simulink model "stabilizer_bar_step35g"  (R2023a)
settings: Solver=ode4  StartTime=0  StopTime=40  FixedStep=Ts_plant  MaxStep=0.001  RelTol=1e-3
InitFcn:
  | run(fullfile(fileparts(get_param(bdroot,'FileName')),'a001_step35g_initialize.m'));
values from neighbouring files (symbols this model uses):
  cycle_cfg = jsondecode(fileread(fullfile(repair_root,'repair_support','repair_cycle_bank.json')))    [a001_step35g_initialize.m]
  entry_cfg = rmfield(entry_bank_source,{'labels','source_hashes','note','source_par_sha256'})    [a001_step35g_initialize.m]
  path_geometry = repair_build_geometry(path_cfg)    [a001_step35g_initialize.m]
  path_Q = [10,0,0;0,10,0;0,0,2]    [a001_step35g_initialize.m]
  path_R = [100,0,0;0,100,0;0,0,10]    [a001_step35g_initialize.m]
  repair_cfg = struct    [a001_step35g_initialize.m]
  repair_simfile = aux_case_cfg.simfile_path    [a001_step35g_initialize.m]
  stadium_cfg = struct('disabled',1)    [a001_step35g_initialize.m]
  state_cfg = profile_cfg.state_protocol    [a001_step35g_initialize.m]
  Ts = 0.01    [a001_step35g_initialize.m]
  Ts_plant = 0.0005    [a001_step35g_initialize.m]
undefined symbols (not defined in the file or in its folder): path_cfg
(part 2 of 2)

== matlab function stabilizer_bar_step35g/路径跟踪层/ContinuousProjection ==
  settings: updateMethod=DISCRETE  sampleTime=Ts
  data: X input; ey output size=1; Y input; psi input; beta input; alignment input size=[3 1]; DeltaChi output size=1; kappa output size=1; diag_project output size=[2 1]; path_geometry parameter; path_cfg parameter
function [ey,DeltaChi,kappa,diag_project] = path_projection(X,Y,psi,beta,alignment,path_geometry,path_cfg)
%#codegen
% 连续Frenet投影：只沿上一个弧长邻域迭代，弧长不取模存储，跨圈不跳点。
% ey为路径左侧正；DeltaChi为实际速度方向psi+beta与投影切向之差。
% 该投影用于式4.10；LQR仍跟踪时间索引参考，二者用途明确区分。
if path_cfg.feedback_enabled==0,ey=0;DeltaChi=0;kappa=0;diag_project=zeros(2,1);return;end
persistent s_prev
if isempty(s_prev),s_prev=0;end
c=cos(alignment(3));sn=sin(alignment(3));
dx=X-alignment(1);dy=Y-alignment(2);
x=c*dx+sn*dy;y=-sn*dx+c*dy;
s=s_prev;
% 牛顿投影的分母即1-kappa*ey；失效时停止，不夹紧分母。
for it=1:12
    [px,py,chi,k]=geometry(s,path_geometry,path_cfg);
    ex=x-px;ey0=y-py;
    lateral=-sin(chi)*ex+cos(chi)*ey0;
    den=1-k*lateral;
    % 分母状态只记录，不触发外加仿真停止。
    ds=(cos(chi)*ex+sin(chi)*ey0)/den;
    % 有界迭代步只用于局部求根，不能切换到全局另一段路径。
    s=s+ds;
    % 投影点跳变由路径误差和CarSim响应体现，不用Assert截断仿真。
    if abs(ds)<1e-7,break;end
end
[px,py,chi,kappa]=geometry(s,path_geometry,path_cfg);
ey=-sin(chi)*(x-px)+cos(chi)*(y-py);
tangential=cos(chi)*(x-px)+sin(chi)*(y-py);
% 切向投影残差保留在后续诊断中。
DeltaChi=atan2(sin(psi+beta-alignment(3)-chi),cos(psi+beta-alignment(3)-chi));
den=1-kappa*ey;
% 分母状态只记录，不触发外加仿真停止。
s_prev=s;diag_project=[s;den];
end
function [x,y,chi,k]=geometry(s,table,cfg)
if (cfg.mode==4 || cfg.mode==5),q=mod(s,cfg.length);else,q=s;end
[x,y,chi]=sample_geometry(q,table,cfg);
[k,~,~,~,~]=repair_path_profile(s,cfg);
end
function [x,y,chi]=sample_geometry(q,table,cfg)
% 均匀节点三次Hermite位置插值，切向由同一曲率积分生成。
ds=table(2,1)-table(1,1);j=min(max(floor(q/ds)+1,1),size(table,1)-1);
h=table(j+1,1)-table(j,1);u=(q-table(j,1))/h;
h00=2*u^3-3*u^2+1;h10=u^3-2*u^2+u;h01=-2*u^3+3*u^2;h11=u^3-u^2;
x=h00*table(j,2)+h10*h*cos(table(j,4))+h01*table(j+1,2)+h11*h*cos(table(j+1,4));
y=h00*table(j,3)+h10*h*sin(table(j,4))+h01*table(j+1,3)+h11*h*sin(table(j+1,4));
[~,~,~,~,chi]=repair_path_profile(q,cfg);
end

function [k,bw,dbds,stage,chi]=repair_path_profile(s,cfg)
% 曲率与侧偏角分别生成；chi是曲率对弧长的解析积分。
% mode=1入漂维持，2同步退出，3先恢复beta再退出，4原操场，5提前恢复beta操场。
L=cfg.transition;R=cfg.R;C=cfg.plateau;
% 普通轨迹：stage=1直线、2入弯、3恒曲率、4出弯、5末直线。
% 曲率与漂移权重独立；mode=6始终bw=0，不能只把beta设零。
if cfg.mode==6
 q=s-cfg.straight;bw=0;dbds=0;
 if q<=0,k=0;chi=0;stage=1;
 elseif q<L
  u=q/L;[h,~]=smooth(u);k=h/R;chi=L/R*primitive(u);stage=2;
 elseif q<L+C,k=1/R;chi=(q-L/2)/R;stage=3;
 elseif q<2*L+C
  u=(q-L-C)/L;[h,~]=smooth(u);k=(1-h)/R;chi=(L/2+C+L*(u-primitive(u)))/R;stage=4;
 else,k=0;chi=(L+C)/R;stage=5;end
 return;
end
if cfg.mode==4 || cfg.mode==5
 q=mod(s,cfg.half)-cfg.straight;half=floor(s/cfg.half);
 if q<=0,k=0;bw=0;dbds=0;stage=1;theta=0;
 elseif q<L
  u=q/L;[bw,db]=smooth(u);dbds=db/L;k=bw/R;stage=2;theta=L/R*primitive(u);
 elseif q<L+C
  k=1/R;bw=1;dbds=0;stage=3;theta=(q-L/2)/R;
  if cfg.mode==5 && q>L+C-L
   u=(q-(L+C-L))/L;[z,dz]=smooth(u);bw=1-z;dbds=-dz/L;stage=4;
  end
 else
  u=min((q-L-C)/L,1);[z,dz]=smooth(u);k=(1-z)/R;
  if cfg.mode==4,bw=1-z;dbds=-dz/L;else,bw=0;dbds=0;end
  stage=4;theta=(L/2+C+L*(u-primitive(u)))/R;
 end
 chi=pi*half+theta;stage=stage+4*mod(half,2);return;
end
% 入漂维持允许曲率与侧偏的建立长度/起点不同；chi仍只由曲率积分确定。
if cfg.mode==1
 q=s-cfg.straight;u=min(max(q/cfg.transition,0),1);[hk,~]=smooth(u);k=hk/cfg.R;
 if q<=0,chi=0;elseif q<cfg.transition,chi=cfg.transition/cfg.R*primitive(u);else,chi=(q-cfg.transition/2)/cfg.R;end
 v=min(max((q-cfg.beta_delay)/cfg.beta_transition,0),1);[bw,db]=smooth(v);dbds=db/cfg.beta_transition;
 if q<=0,stage=1;elseif u<1||v<1,stage=2;else,stage=3;end
 return;
end
q=s-cfg.straight;
if q<=0,k=0;bw=0;dbds=0;stage=1;chi=0;return;end
if q<L
 u=q/L;[bw,db]=smooth(u);dbds=db/L;k=bw/R;stage=2;chi=L/R*primitive(u);return;
end
k=1/R;bw=1;dbds=0;stage=3;chi=(q-L/2)/R;
if cfg.mode==1,return;end
% 独立退出站点由已通过3s稳态门槛的前置试验给出，不猜测稳定起点。
e=s-cfg.exit_s;if e<0,return;end
if cfg.mode==2
 u=min(e/L,1);[z,dz]=smooth(u);k=(1-z)/R;bw=1-z;dbds=-dz/L;
 chi=(cfg.exit_s-cfg.straight-L/2+L*(u-primitive(u)))/R;stage=4;
else
 u=min(e/L,1);[z,dz]=smooth(u);bw=1-z;dbds=-dz/L;stage=4;
 if e>=L
  z2=min((e-L)/L,1);[h,~]=smooth(z2);k=(1-h)/R;
  chi=(cfg.exit_s+L-cfg.straight-L/2+L*(z2-primitive(z2)))/R;stage=5;
 end
end
end
function [h,dh]=smooth(u)
h=10*u^3-15*u^4+6*u^5;dh=30*u^2*(1-u)^2;
end
function v=primitive(u)
v=2.5*u^4-3*u^5+u^6;
end

== matlab function stabilizer_bar_step35g/CarSimInterface/FrontWheelActuator ==
  settings: updateMethod=DISCRETE  sampleTime=Ts_plant
  data: target input; left output; right output; left_rate output; right_rate output; diag output size=[6 1]; repair_cfg parameter
function [left,right,left_rate,right_rate,diag] = steer_direct(target,repair_cfg)
% 直接前轮输入，不叠加外部转角幅值或速率限制；角速度同步记录指令变化率。
persistent previous
if isempty(previous),previous=0;end
angle=target(1);
if repair_cfg.entry_mode==1,limit=repair_cfg.entry_steer_rate*repair_cfg.Ts_plant;angle=min(max(angle,previous-limit),previous+limit);end
rate=(angle-previous)/repair_cfg.Ts_plant;previous=angle;
left=angle*180/pi;right=left;left_rate=rate*180/pi;right_rate=left_rate;
diag=[angle;angle;angle;rate;0;0];
end

== matlab function stabilizer_bar_step35g/CarSimInterface/InterfaceTestSelector ==
  settings: updateMethod=DISCRETE  sampleTime=Ts_plant
  data: command input size=[8 1]; u output size=[8 1]; t input; repair_interface_test parameter
function u=interface_selector(command,t,repair_interface_test)
% 仅在显式接口验证中产生2deg、10deg/s分段线性转角；其余时候透传。
u=command;
if repair_interface_test==0,return;end
knots=[0,.4,.6,.9,1.1,1.3,1.6,1.8,2,2.3,2.7,3,3.2,3.6];
left=[0,0,2,2,0,0,0,0,2,2,-2,-2,0,0];right=[0,0,0,0,0,-2,-2,0,2,2,-2,-2,0,0];
j=1;for k=1:13,if t>=knots(k),j=k;end;end
q=min(max((t-knots(j))/(knots(j+1)-knots(j)),0),1);
lr=(left(j+1)-left(j))/(knots(j+1)-knots(j));rr=(right(j+1)-right(j))/(knots(j+1)-knots(j));
u=[left(j)+q*(left(j+1)-left(j));right(j)+q*(right(j+1)-right(j));lr;rr;0;0;0;0];
end

== matlab function stabilizer_bar_step35g/StageStop ==
  settings: updateMethod=DISCRETE  sampleTime=Ts
  data: valid input; stop output; plant input size=[50 1]; repair_interface_test parameter
function stop=stage_stop(valid,plant,repair_interface_test)
% 仅保留信号记录；候选、轮荷、查表告警不再触发自定义Stop Simulation。
stop=0;
end

== matlab function stabilizer_bar_step35g/路径跟踪层/ReferenceAlignment ==
  settings: updateMethod=DISCRETE  sampleTime=Ts
  data: t input; ref output size=[14 1]; X input; Y input; psi input; V input; alignment output size=[3 1]; path_geometry parameter; path_cfg parameter
function [ref,alignment]=stadium_reference(t,X,Y,psi,V,path_geometry,path_cfg)
% 统一工况参考：初始实际质心对齐；入漂维持与两种退出独立选择。
% ref的14项接口与现有路径层保持一致，所有角度为rad。
persistent origin initial_speed
if isempty(origin),origin=[X;Y;psi];initial_speed=V;end
alignment=origin;T=path_cfg.ramp_time;u=min(max(t/T,0),1);H=10*u^3-15*u^4+6*u^5;
Vr=initial_speed+(path_cfg.V-initial_speed)*H;
if t<=T,s=initial_speed*t+(path_cfg.V-initial_speed)*T*(2.5*u^4-3*u^5+u^6);
else,s=(initial_speed+path_cfg.V)*T/2+path_cfg.V*(t-T);end
[k,bw,dbds,stage,chi]=repair_path_profile(s,path_cfg);
beta=path_cfg.beta*bw;bdot=path_cfg.beta*dbds*Vr;
if (path_cfg.mode==4 || path_cfg.mode==5),q=mod(s,path_cfg.length);lap=floor(s/path_cfg.length);else,q=s;lap=0;end
[x,y,~]=sample_geometry(q,path_geometry,path_cfg);
c=cos(origin(3));sn=sin(origin(3));chi=chi+origin(3);
ref=[origin(1)+c*x-sn*y;origin(2)+sn*x+c*y;chi-beta;Vr*cos(beta);Vr*sin(beta); ...
 k*Vr-bdot;Vr;beta;k;bw;stage;lap;s;chi];
end

function [x,y,chi]=sample_geometry(q,table,cfg)
% 均匀节点三次Hermite位置插值，切向由同一曲率积分生成。
ds=table(2,1)-table(1,1);j=min(max(floor(q/ds)+1,1),size(table,1)-1);
h=table(j+1,1)-table(j,1);u=(q-table(j,1))/h;
h00=2*u^3-3*u^2+1;h10=u^3-2*u^2+u;h01=-2*u^3+3*u^2;h11=u^3-u^2;
x=h00*table(j,2)+h10*h*cos(table(j,4))+h01*table(j+1,2)+h11*h*cos(table(j+1,4));
y=h00*table(j,3)+h10*h*sin(table(j,4))+h01*table(j+1,3)+h11*h*sin(table(j+1,4));
[~,~,~,~,chi]=repair_path_profile(q,cfg);
end

function [k,bw,dbds,stage,chi]=repair_path_profile(s,cfg)
% 曲率与侧偏角分别生成；chi是曲率对弧长的解析积分。
% mode=1入漂维持，2同步退出，3先恢复beta再退出，4原操场，5提前恢复beta操场。
L=cfg.transition;R=cfg.R;C=cfg.plateau;
% 普通轨迹：stage=1直线、2入弯、3恒曲率、4出弯、5末直线。
% 曲率与漂移权重独立；mode=6始终bw=0，不能只把beta设零。
if cfg.mode==6
 q=s-cfg.straight;bw=0;dbds=0;
 if q<=0,k=0;chi=0;stage=1;
 elseif q<L
  u=q/L;[h,~]=smooth(u);k=h/R;chi=L/R*primitive(u);stage=2;
 elseif q<L+C,k=1/R;chi=(q-L/2)/R;stage=3;
 elseif q<2*L+C
  u=(q-L-C)/L;[h,~]=smooth(u);k=(1-h)/R;chi=(L/2+C+L*(u-primitive(u)))/R;stage=4;
 else,k=0;chi=(L+C)/R;stage=5;end
 return;
end
if cfg.mode==4 || cfg.mode==5
 q=mod(s,cfg.half)-cfg.straight;half=floor(s/cfg.half);
 if q<=0,k=0;bw=0;dbds=0;stage=1;theta=0;
 elseif q<L
  u=q/L;[bw,db]=smooth(u);dbds=db/L;k=bw/R;stage=2;theta=L/R*primitive(u);
 elseif q<L+C
  k=1/R;bw=1;dbds=0;stage=3;theta=(q-L/2)/R;
  if cfg.mode==5 && q>L+C-L
   u=(q-(L+C-L))/L;[z,dz]=smooth(u);bw=1-z;dbds=-dz/L;stage=4;
  end
 else
  u=min((q-L-C)/L,1);[z,dz]=smooth(u);k=(1-z)/R;
  if cfg.mode==4,bw=1-z;dbds=-dz/L;else,bw=0;dbds=0;end
  stage=4;theta=(L/2+C+L*(u-primitive(u)))/R;
 end
 chi=pi*half+theta;stage=stage+4*mod(half,2);return;
end
% 入漂维持允许曲率与侧偏的建立长度/起点不同；chi仍只由曲率积分确定。
if cfg.mode==1
 q=s-cfg.straight;u=min(max(q/cfg.transition,0),1);[hk,~]=smooth(u);k=hk/cfg.R;
 if q<=0,chi=0;elseif q<cfg.transition,chi=cfg.transition/cfg.R*primitive(u);else,chi=(q-cfg.transition/2)/cfg.R;end
 v=min(max((q-cfg.beta_delay)/cfg.beta_transition,0),1);[bw,db]=smooth(v);dbds=db/cfg.beta_transition;
 if q<=0,stage=1;elseif u<1||v<1,stage=2;else,stage=3;end
 return;
end
q=s-cfg.straight;
if q<=0,k=0;bw=0;dbds=0;stage=1;chi=0;return;end
if q<L
 u=q/L;[bw,db]=smooth(u);dbds=db/L;k=bw/R;stage=2;chi=L/R*primitive(u);return;
end
k=1/R;bw=1;dbds=0;stage=3;chi=(q-L/2)/R;
if cfg.mode==1,return;end
% 独立退出站点由已通过3s稳态门槛的前置试验给出，不猜测稳定起点。
e=s-cfg.exit_s;if e<0,return;end
if cfg.mode==2
 u=min(e/L,1);[z,dz]=smooth(u);k=(1-z)/R;bw=1-z;dbds=-dz/L;
 chi=(cfg.exit_s-cfg.straight-L/2+L*(u-primitive(u)))/R;stage=4;
else
 u=min(e/L,1);[z,dz]=smooth(u);bw=1-z;dbds=-dz/L;stage=4;
 if e>=L
  z2=min((e-L)/L,1);[h,~]=smooth(z2);k=(1-h)/R;
  chi=(cfg.exit_s+L-cfg.straight-L/2+L*(z2-primitive(z2)))/R;stage=5;
 end
end
end
function [h,dh]=smooth(u)
h=10*u^3-15*u^4+6*u^5;dh=30*u^2*(1-u)^2;
end
function v=primitive(u)
v=2.5*u^4-3*u^5+u^6;
end

== matlab function stabilizer_bar_step35g/EntryLocalMode/EntryLocalControl ==
  settings: updateMethod=DISCRETE  sampleTime=Ts
  data: y input size=[50 1]; command output size=[5 1]; t input; diag output size=[70 1]; entry_cfg parameter; repair_cfg parameter; cycle_diag output size=[16 1]; cycle_cfg parameter; stadium_packet input; state_cfg parameter
function [command,diag,cycle_diag]=cycle_control(y,t,entry_cfg,repair_cfg,cycle_cfg,stadium_packet,state_cfg)
%#codegen
% 无路径任务：时间参考→五状态反馈→原公共执行层。这里不读取XY/曲率/方向。
% y是CarSim原50路，轮序FL/FR/RL/RR；stadium_packet现只输送原生600点事件。
% Roll/AVx仅用于原物理接管，K只乘[V,beta,AVz,kappa_f,kappa_r]。
% 进入固定10s维持后不回退/重计；误差与退出门控分开，失败也保留退漂证据。
persistent phase readyTime elapsed entryStart captureTime satTime mixStart holdStart exitStart straightCapture straightMix previousRef refInitialized vprev wprev initialized protection
if isempty(initialized)
 phase=0;readyTime=0;elapsed=0;entryStart=0;captureTime=0;satTime=0;mixStart=0;holdStart=0;exitStart=0;straightCapture=0;straightMix=0;
 previousRef=zeros(7,1);refInitialized=false;vprev=zeros(3,1);wprev=zeros(4,1);initialized=false;protection=false;
end
command=zeros(5,1);diag=zeros(70,1);cycle_diag=zeros(16,1);
Ts=repair_cfg.Ts;Rw=repair_cfg.Rw;Iw=repair_cfg.Iw;
x=[hypot(y(2),y(3))/3.6;y(4)*pi/180;y(5)*pi/180;mean(y(27:28));mean(y(29:30));y(8)*pi/180;y(26)*pi/180];
omega=y(21:24)*pi/30;Fz=y(17:20);last=entry_cfg.nodes(end);
assert(all(isfinite(x))&&all(isfinite(Fz)),'Nonfinite state or wheel load');first=~initialized;
if first,vprev=entry_cfg.normal.v;wprev=omega;initialized=true;end
elapsed=elapsed+Ts;if protection,satTime=satTime+Ts;else,satTime=0;end
inside=all(abs(x-last.x)<=entry_cfg.thresholds)&&all(Fz>0)&&satTime<.2;
progress=0;mix=0;weight=0;holdTime=0;exitProgress=0;substage=0;exitElapsed=0;holdgate=false;prepareFailed=false;
ref=entry_cfg.normal;
% 准备仍由实际直行状态持续1s确定，不使用道路站点或世界坐标。
if phase==0
 ready=abs(x(1)-12)<=.2&&abs(x(2))<=pi/180&&abs(x(3))<=.02;
 if ready,readyTime=readyTime+Ts;else,readyTime=0;end
 ref=mixnode(entry_cfg.normal,entry_cfg.nodes(1),smooth5(t/2));
 if readyTime>=1-1e-9&&elapsed<10,phase=1;entryStart=t;elseif elapsed>=10,prepareFailed=true;end
end
if phase>=1&&phase<=3
 q=max(0,t-entryStart);progress=min(q/state_cfg.entry_reference_s,1);
 % 连续经过节点：预加载复用原公式；其后β一次平滑到−30°。
 % β同时作为原银行的调度坐标，x/v/K/offset共享一个插值比例。
 if q<state_cfg.preload_end_s
  ref=sampleNodes(entry_cfg.nodes(1:7),entry_cfg.grid,smooth5(q/state_cfg.prefix_s));
 else
  h=smooth5((q-state_cfg.preload_end_s)/(state_cfg.entry_reference_s-state_cfg.preload_end_s));
  beta=(1-h)*entry_cfg.nodes(3).x(2)+h*entry_cfg.nodes(9).x(2);
  j=3;
  for k=3:8
   if beta<=entry_cfg.nodes(k).x(2),j=k;end
  end
  f=(beta-entry_cfg.nodes(j).x(2))/(entry_cfg.nodes(j+1).x(2)-entry_cfg.nodes(j).x(2));
  ref=mixnode(entry_cfg.nodes(j),entry_cfg.nodes(j+1),min(max(f,0),1));
 end
 if phase==1
  if inside,captureTime=captureTime+Ts;else,captureTime=0;end
  % 原七项物理接管+独立600原生点确认；原生事件由快采样块生成。
  if q>=state_cfg.entry_reference_s-1e-9&&captureTime>=.3-1e-9&&stadium_packet(1)>0.5
   phase=2;mixStart=t;
  end
 end
 if phase==2
  mix=smooth5((t-mixStart)/state_cfg.handover_s);ref=mixnode(ref,last,mix);
  if t-mixStart>=state_cfg.handover_s-1e-9,phase=3;holdStart=t;end
 end
 if phase==3
  ref=last;mix=1;holdTime=max(0,t-holdStart);
  % 固定窗口满10s即退漂；不以较好的末段RMSE来推迟或重开窗口。
  if holdTime>=state_cfg.maintain_s-1e-9,phase=4;exitStart=t;holdgate=true;end
 end
 weight=mix;
end
if phase>=4
 exitElapsed=max(0,t-exitStart);exitProgress=min(exitElapsed/state_cfg.exit_reference_s,1);
 if exitElapsed<state_cfg.exit_to15_s
  substage=1;ref=mixnode(cycle_cfg.nodes(1),cycle_cfg.nodes(2),smooth5(exitElapsed/state_cfg.exit_to15_s));
 elseif exitElapsed<state_cfg.exit_to15_s+state_cfg.exit_to10_s
  substage=2;ref=mixnode(cycle_cfg.nodes(2),cycle_cfg.nodes(3),smooth5((exitElapsed-state_cfg.exit_to15_s)/state_cfg.exit_to10_s));
 else
  substage=3;q=min((exitElapsed-state_cfg.exit_to15_s-state_cfg.exit_to10_s)/state_cfg.exit_legacy_s,1);
  if q<.5,p=.5*smooth5(2*q);else,p=.5+.5*smooth5(2*q-1);end
  ref=sampleNodes(cycle_cfg.nodes(3:7),cycle_cfg.grid,p);
 end
 normal=cycle_cfg.nodes(end);
 inside=all(abs(x-normal.x)<=cycle_cfg.straight_capture)&&all(Fz>0)&&~protection&&exitProgress>=1-1e-8;
 if inside,straightCapture=straightCapture+Ts;else,straightCapture=0;end
 if phase==4&&straightCapture>=.3-1e-9,phase=5;straightMix=0;end
 if phase==5,straightMix=min(1,straightMix+Ts/.5);if straightMix>=1-1e-9,phase=6;end,end
 weight=0;if phase==5,weight=smooth5(straightMix);elseif phase==6,weight=1;end
 ref=mixnode(ref,normal,weight);
end
request=ref.v-feedback_delta(ref.K,x-ref.x);
rates=zeros(7,1);if refInitialized,rates=(ref.x-previousRef)/Ts;end;previousRef=ref.x;refInitialized=true;
cycle_diag=[phase;exitProgress;substage;holdTime;double(holdgate);double(inside);straightCapture;weight;exitElapsed;rates];
% 公共执行层：真实接地点速度、实际Fx负载补偿与冻结的局部执行预算。
lo=[ref.v(1)-entry_cfg.steer_deviation;entry_cfg.slip_low];hi=[ref.v(1)+entry_cfg.steer_deviation;entry_cfg.slip_high];
v=min(max(request,lo),hi);slew=[entry_cfg.steering_rate_rad_s;entry_cfg.slip_rate;entry_cfg.slip_rate];v=min(max(v,vprev-slew*Ts),vprev+slew*Ts);vprev=v;
contact=Rw*omega./(1+y(27:30));assert(all(isfinite(contact))&&all(contact>0),'Invalid contact velocity');
candidate=contact/Rw.*(1+[v(2);v(2);v(3);v(3)]);loadTorque=Rw*y(9:12)+ref.offset;kw=entry_cfg.wheel_kw;
if first,wd=omega;dwd=zeros(4,1);
else
 gain=kw+Iw/Ts;low=(-entry_cfg.torque_limit+kw*omega+Iw/Ts*wprev-loadTorque)/gain;high=(entry_cfg.torque_limit+kw*omega+Iw/Ts*wprev-loadTorque)/gain;
 low=max(low,wprev-entry_cfg.omega_acceleration*Ts);high=min(high,wprev+entry_cfg.omega_acceleration*Ts);assert(all(low<=high),'Empty torque and wheel acceleration budget');
 wd=min(max(candidate,low),high);dwd=(wd-wprev)/Ts;
end
feedback=kw*(wd-omega);inertia=Iw*dwd;raw=feedback+inertia+loadTorque;T=min(max(raw,-entry_cfg.torque_limit),entry_cfg.torque_limit);wprev=wd;
protection=any(abs(T)>=entry_cfg.torque_limit-1e-6);command=[v(1);T];
diag=[phase;progress;mix;double(inside);double(prepareFailed);readyTime;captureTime;satTime;x;ref.x;ref.v;request;v;candidate;wd;omega;feedback;inertia;loadTorque;raw;T;double(any(abs(v-request)>1e-9));double(any(abs(wd-candidate)>1e-9));double(protection);contact];
end
function h=smooth5(q)
q=min(max(q,0),1);h=10*q^3-15*q^4+6*q^5;
end
function out=mixnode(a,b,f)
out=a;out.x=(1-f)*a.x+f*b.x;out.v=(1-f)*a.v+f*b.v;out.K=(1-f)*a.K+f*b.K;out.offset=(1-f)*a.offset+f*b.offset;
end
function out=sampleNodes(nodes,grid,s)
j=1;for k=1:numel(grid)-1,if s>=grid(k),j=k;end,end
f=(s-grid(j))/(grid(j+1)-grid(j));out=mixnode(nodes(j),nodes(j+1),f);
end


function du=feedback_delta(K,error)
% 五项误差反馈：车辆侧倾仍存在，但不直接进入转角/滑移请求。
% K为3×5，状态前五项顺序为V、beta、AVz、前后轴滑移。
du=K*error(1:5);
end

== matlab function stabilizer_bar_step35g/EntryModeSelector ==
  data: newcmd input size=[5 1]; angle output; oldcmd input size=[5 1]; tfl output; tfr output; trl output; trr output; repair_cfg parameter
function [angle,tfl,tfr,trl,trr]=select_commands(newcmd,oldcmd,repair_cfg)
% 模式开关只选择执行输入；不改变两支路的数学公式。
c=oldcmd;if repair_cfg.entry_mode==1,c=newcmd;end
angle=c(1);tfl=c(2);tfr=c(3);trl=c(4);trr=c(5);
end

== matlab function stabilizer_bar_step35g/EntryLocalMode/EntryForceDiagnostic ==
  settings: updateMethod=DISCRETE  sampleTime=Ts
  data: y input size=[50 1]; out output size=[20 1]; diag input size=[70 1]; repair_cfg parameter
function out=entry_force_diagnostic(y,diag,repair_cfg)
%#codegen
% 本块仅记录原三自由度逆解回代及其与实际轮胎合力的差异，不参与执行指令。
% out=[原请求4;代数回代残差3;实际轴力4;实际平面合力矩3;请求平面合力矩3;差值3]。
% 实际合力矩使用四轮Fx/Fy、前轮实测角及轮距；未包含回正力矩/外倾/三维悬架作用。
persistent history initialized
if isempty(initialized),history=zeros(4,1);initialized=false;end
out=zeros(20,1);if repair_cfg.entry_mode==0,return;end
V=diag(9);beta=diag(10);r=diag(11);ref=diag(16:18);Ts=repair_cfg.Ts;
bd=ref(2);rd=ref(3);diffs=zeros(4,1);
if initialized,diffs=([bd;beta;rd;r]-history)/Ts;end
history=[bd;beta;rd;r];initialized=true;
vdot=repair_cfg.k_V*(ref(1)-V);betadot=repair_cfg.k_beta_p*(bd-beta)+repair_cfg.k_beta_d*(diffs(1)-diffs(2));
rdot=repair_cfg.k_r_p*(rd-r)+repair_cfg.k_r_d*(diffs(3)-diffs(4));q=betadot+r;
m=repair_cfg.m;Iz=repair_cfg.Iz;a=repair_cfg.a;b=repair_cfg.b;L=a+b;
angles=[y(38:39)*pi/180;0;0];delta=mean(angles(1:2));cd=cos(delta);sd=sin(delta);
Fxf=m*vdot;Fyr=(-Iz*rdot+a*m*V*q*cos(beta)+a*m*vdot*sin(beta))/L;
Fyf=(Iz*rdot-L*Fxf*sd+b*m*V*q*cos(beta)+b*m*vdot*sin(beta))/(L*cd);
Fxr=(-L*Fxf+Iz*rdot*sd-a*m*V*q*sin(beta)*cd-b*m*V*q*sin(beta-delta)+a*m*vdot*cos(beta)*cd+b*m*vdot*cos(beta-delta))/(L*cd);
bx=Fxf*cd-Fyf*sd+Fxr;by=Fxf*sd+Fyf*cd+Fyr;mz=a*(Fxf*sd+Fyf*cd)-b*Fyr;
back=[(bx*cos(beta)+by*sin(beta))/m;(-bx*sin(beta)+by*cos(beta))/(m*V)-r;mz/Iz];
Fx=y(9:12);Fy=y(13:16);cx=Fx.*cos(angles)-Fy.*sin(angles);cy=Fx.*sin(angles)+Fy.*cos(angles);
actual=[sum(cx);sum(cy);a*sum(cy(1:2))-b*sum(cy(3:4))+repair_cfg.d/2*(cx(2)-cx(1)+cx(4)-cx(3))];
request=[bx;by;mz];out=[Fxf;Fyf;Fxr;Fyr;back-[vdot;betadot;rdot];sum(Fx(1:2));sum(Fy(1:2));sum(Fx(3:4));sum(Fy(3:4));actual;request;actual-request];
end

== matlab function stabilizer_bar_step35g/路径跟踪层/StadiumGuidance ==
  settings: updateMethod=DISCRETE  sampleTime=Ts_plant
  data: y input; packet output; t input; stadium_diag output; stadium_cfg parameter; entry_cfg parameter; repair_cfg parameter; roll_feedback output; feedback_diag output; state_cfg parameter
function [packet,stadium_diag,roll_feedback,feedback_diag]=stadium_guidance(y,t,stadium_cfg,entry_cfg,repair_cfg,state_cfg)
%#codegen
% 原操场模块现为独立原生事件检查：0.0005s每点计算，不投影/纠偏。
% packet19仅前5项有意义：已确认、确认时刻、合格段起点、计数、当前合格。
% 通过0.01s采样传给阶段调度；600点事件时刻仍保存原生精度。
% 旧输出尺寸保持：stadium_diag17全零，roll_feedback6物理诊断，feedback_diag17。
persistent count latched confirm eventStart lastIndex
if isempty(count),count=0;latched=false;confirm=-1;eventStart=-1;lastIndex=-1;end
packet=zeros(19,1);stadium_diag=zeros(17,1);roll_feedback=zeros(6,1);feedback_diag=zeros(17,1);
x=[hypot(y(2),y(3))/3.6;y(4)*pi/180;y(5)*pi/180];
inside=all(abs(x-state_cfg.target)<=state_cfg.entry_tolerance)&&x(3)>0;
index=round(t/state_cfg.native_step_s);
if index>lastIndex
 assert(index==lastIndex+1,'Native entry event missed 0.0005s sample');
 if inside,count=count+1;else,count=0;end
 if count==state_cfg.entry_samples&&~latched
  latched=true;confirm=t;eventStart=t-(state_cfg.entry_samples-1)*state_cfg.native_step_s;
 end
 lastIndex=index;
end
packet(1:5)=[double(latched);confirm;eventStart;count;double(inside)];
roll_feedback=[y(8)*pi/180;y(26)*pi/180;0;0;0;0];
feedback_diag(1:12)=[count;double(inside);double(latched);eventStart;confirm;index;x;state_cfg.target];
end

== matlab function stabilizer_bar_step35g/ActiveRollResearch/MomentDemand ==
  settings: updateMethod=DISCRETE  sampleTime=Ts_plant
  data: raw input; phi output; rate output; moment output; dk output; asb_cfg parameter; t input; dm output
function [phi,rate,moment,dk,dm]=asb_pulse_moment(raw,asb_cfg,t)
%#codegen
% 固定时窗开环力矩 / Timed Open-loop Moment。
% raw为原26路悬架输出，phi/rate仅供机械诊断；不参与力矩决策。
% moment前/后轴单位Nm；正值指左正、右负的轮端等反向力偶。
% 在冻结基线的时窗内保持固定力矩，0.10s余弦边沿用于避免阶跃。
assert(all(isfinite(raw)),'ASB:Nonfinite suspension measurement');
phi=raw(1:2)*pi/180;rate=raw(3:4)*pi/180;
dk=zeros(2,1); % 没有辅助刚度或状态反馈；内部原384/384稳定杆仍在车辆模型中。
g=0;dg=0;lo=asb_cfg.pulse_start_s;hi=asb_cfg.pulse_end_s;edge=asb_cfg.pulse_edge_s;
if t>lo && t<hi
    if t<lo+edge
        q=(t-lo)/edge;g=(1-cos(pi*q))/2;dg=pi*sin(pi*q)/(2*edge);
    elseif t>hi-edge
        q=(hi-t)/edge;g=(1-cos(pi*q))/2;dg=-pi*sin(pi*q)/(2*edge);
    else
        g=1;
    end
end
moment=asb_cfg.pulse_moment_Nm*g;
dm=asb_cfg.pulse_moment_Nm*dg; % 力矩变化率为指令解析导数，仅用于日志。
end

== matlab function stabilizer_bar_step35g/ActiveRollResearch/ForcePair ==
  settings: updateMethod=DISCRETE  sampleTime=Ts_plant
  data: raw input; forces output; phi input; rate input; moment input; dk input; diag output; asb_cfg parameter; dm input
function [forces,diag]=asb_pulse_force(raw,phi,rate,moment,dk,asb_cfg,dm)
%#codegen
% 轮端力偶到弹簧附加力 / Wheel Couple to Spring Force。
% 内部轮序FL FR RL RR；GUI排列仍由原Selector转为L1 L2 R1 R2。
% 原物理映射不变：正FsExt为弹簧压缩力，运动比前0.959、后0.797。
% q=M/lever，左右轮端分别+q/-q；每轴轮端合力为零。
lever=asb_cfg.track_m-[sum(raw(21:22));sum(raw(23:24))]*.001;
assert(all(lever>0)&&all(isfinite(moment)),'ASB:Invalid force-couple geometry');
q=moment./lever;wheel=[q(1);-q(1);q(2);-q(2)];forces=wheel./asb_cfg.motion_ratio;
% 实际接收的FsExt用于回查，不能用指令冒充车辆收到的力矩。
actual=raw(5:8);actualWheel=actual.*asb_cfg.motion_ratio;
actualMoment=[(actualWheel(1)-actualWheel(2))*lever(1)/2;(actualWheel(3)-actualWheel(4))*lever(2)/2];
net=[sum(actualWheel(1:2));sum(actualWheel(3:4))];
power=moment.*rate;jrate=raw(13:16)*.001;
powerSpring=-[sum(actualWheel(1:2).*jrate(1:2));sum(actualWheel(3:4).*jrate(3:4))];
geometricPhi=atan2([raw(10)-raw(9);raw(12)-raw(11)]*.001,lever);
% 保持44路布局；35:36改为真实开环力矩指令导数dm，3:4仍为零辅助刚度。
diag=[phi;rate;dk;moment;actualMoment;actualMoment-moment;lever;wheel;forces;actual;net;power;powerSpring;powerSpring-power;dm;geometricPhi;geometricPhi-phi;raw(25:26);asb_cfg.target_K_deg];
end

== matlab function stabilizer_bar_step35g/MATLAB Function ==
  settings: updateMethod=DISCRETE  sampleTime=Ts
  data: Vx input; V output; Vy input
function V = cg_speed(Vx,Vy)
%#codegen
V = hypot(Vx,Vy);
end

== matlab function stabilizer_bar_step35g/路径跟踪层/PoseError ==
  settings: updateMethod=DISCRETE  sampleTime=Ts
  data: X input; xi output size=[3 1]; Y input; psi input; ref input size=[14 1]
function xi = pose_error(X,Y,psi,ref)
%#codegen
% 论文式4.4~4.8：全局位置误差为实际减参考，航向误差取主值。
% 参考psi保持连续累积，只有相对误差wrap，避免参考跨圈跳变。
xi=[X-ref(1);Y-ref(2);atan2(sin(psi-ref(3)),cos(psi-ref(3)))];
end

== matlab function stabilizer_bar_step35g/路径跟踪层/OnlineLQR ==
  settings: updateMethod=DISCRETE  sampleTime=Ts
  data: ref input size=[14 1]; desired output size=[3 1]; xi input size=[3 1]; diag_lqr output size=[11 1]; path_Q parameter; path_R parameter; path_cfg parameter
function [desired,diag_lqr] = path_lqr(ref,xi,path_Q,path_R,path_cfg)
% 在线LQR目标直接输出；CARE残差保留诊断，不触发自定义Assert停止。
if path_cfg.feedback_enabled==0,desired=ref(4:6);diag_lqr=zeros(11,1);return;end
coder.extrinsic('lqr');c=cos(ref(3));s=sin(ref(3));vx=ref(4);vy=ref(5);
A=[0,0,-vx*s-vy*c;0,0,vx*c-vy*s;0,0,0];B=[c,-s,0;s,c,0;0,0,1];
K=zeros(3);P=zeros(3);[K,P]=lqr(A,B,path_Q,path_R);
AP=A'*P+P*A;PB=P*B*(path_R\(B'*P));
res=norm(AP-PB+path_Q,'fro')/(1+norm(AP,'fro')+norm(PB,'fro')+norm(path_Q,'fro'));
desired=ref(4:6)-K*xi;ok=all(isfinite(K(:)))&&isfinite(res)&&res<=path_cfg.care_tol;
diag_lqr=[K(:);res;double(ok)];
end

== matlab function stabilizer_bar_step35g/车辆运动控制层/StateFeasibility ==
  settings: updateMethod=DISCRETE  sampleTime=Ts
  data: actual input size=[3 1]; packet output size=[13 1]; desired input size=[3 1]; delta input; loads input size=[2 1]; blend input; path input size=[3 1]; omega input size=[4 1]; contact input size=[8 1]; accepted output size=[3 1]; diag output size=[134 1]; valid output; repair_cfg parameter
function [packet,accepted,diag,valid] = state_governor(actual,desired,delta,loads,blend,path,omega,contact,repair_cfg)
% 直接把完整LQR状态参考送入原状态控制律，不做可行候选搜索或指令缩放。
% actual=[V;beta;r]，desired=[Vx_d;Vy_d;r_d]，path=[e_y;DeltaChi;kappa]；SI单位。
% 轮胎力可达性和执行器响应交由CarSim输出反映；diag只记录直通状态。
persistent history initialized
if isempty(initialized),history=zeros(4,1);initialized=false;end
V=actual(1);beta=actual(2);r=actual(3);
Vd=hypot(desired(1),desired(2));beta_d=atan2(desired(2),desired(1));r_d=desired(3);
eV=Vd-V;eBeta=atan2(sin(beta_d-beta),cos(beta_d-beta));eR=r_d-r;
if initialized
    beta_d_dot=atan2(sin(beta_d-history(1)),cos(beta_d-history(1)))/repair_cfg.Ts;
    beta_dot=atan2(sin(beta-history(2)),cos(beta-history(2)))/repair_cfg.Ts;
    r_d_dot=(r_d-history(3))/repair_cfg.Ts;r_dot=(r-history(4))/repair_cfg.Ts;
else
    beta_d_dot=0;beta_dot=0;r_d_dot=0;r_dot=0;
end
den=1-path(3)*path(1);
beta_cmd=repair_cfg.k_beta_p*eBeta+repair_cfg.k_beta_d*(beta_d_dot-beta_dot)+ ...
    repair_cfg.k_beta*path(3)*V*cos(path(2))/den;
r_cmd=repair_cfg.k_r_p*eR+repair_cfg.k_r_d*(r_d_dot-r_dot);
V_cmd=repair_cfg.k_V*eV;
packet=[Vd;beta_d;r_d;eV;eBeta;eR;beta_cmd;r_cmd;V_cmd;beta_d_dot;beta_dot;r_d_dot;r_dot];
accepted=desired;
valid=all(isfinite([actual;desired;delta;loads;blend;path;omega;contact;packet]));
diag=nan(134,1);diag(1)=1;diag(2)=double(valid);diag(3)=1;diag(4)=NaN;diag(5)=1;
diag(6:8)=desired;diag(9:11)=accepted;diag(100)=double(~valid);diag(101)=0;
history=[beta_d;beta;r_d;r];initialized=true;
end

== matlab function stabilizer_bar_step35g/车辆运动控制层/RawDynamicsInverse ==
  settings: updateMethod=DISCRETE  sampleTime=Ts
  data: packet input size=[13 1]; F output size=[4 1]; delta input; Fzr input; blend input; actual input size=[3 1]; status output; repair_cfg parameter; residual output size=[3 1]
function [F,status,residual] = inverse_block(packet,delta,Fzr,blend,actual,repair_cfg)
% 三自由度动力学逆解输出未裁剪的轴级目标力，残差仅记录、不阻止执行。
qd=packet(7)+actual(3);V=actual(1);beta=actual(2);rdot=packet(8);Vdot=packet(9);
Fxf=repair_cfg.m*Vdot;cd=cos(delta);sd=sin(delta);L=repair_cfg.a+repair_cfg.b;
Fyr=(-repair_cfg.Iz*rdot+repair_cfg.a*repair_cfg.m*V*qd*cos(beta)+ ...
    repair_cfg.a*repair_cfg.m*Vdot*sin(beta))/L;
Fyf=(repair_cfg.Iz*rdot-L*Fxf*sd+repair_cfg.b*repair_cfg.m*V*qd*cos(beta)+ ...
    repair_cfg.b*repair_cfg.m*Vdot*sin(beta))/(L*cd);
Fxr=(-L*Fxf+repair_cfg.Iz*rdot*sd-repair_cfg.a*repair_cfg.m*V*qd*sin(beta)*cd- ...
    repair_cfg.b*repair_cfg.m*V*qd*sin(beta-delta)+repair_cfg.a*repair_cfg.m*Vdot*cos(beta)*cd+ ...
    repair_cfg.b*repair_cfg.m*Vdot*cos(beta-delta))/(L*cd);
F=[Fxf;Fyf;Fxr;Fyr];bx=F(1)*cd-F(2)*sd+F(3);by=F(1)*sd+F(2)*cd+F(4);
Vdot_back=(bx*cos(beta)+by*sin(beta))/repair_cfg.m;
beta_dot_back=(-bx*sin(beta)+by*cos(beta))/(repair_cfg.m*V)-actual(3);
r_dot_back=(repair_cfg.a*(F(1)*sd+F(2)*cd)-repair_cfg.b*F(4))/repair_cfg.Iz;
residual=[Vdot_back-packet(9);beta_dot_back-packet(7);r_dot_back-packet(8)];
status=int8(0); %#ok<NASGU> 保留原状态端口，力能否实现以CarSim实际响应判断。
end

== matlab function stabilizer_bar_step35g/车辆运动控制层/ForceCorrection ==
  settings: updateMethod=DISCRETE  sampleTime=Ts
  data: F input size=[4 1]; alpha output; actual input size=[3 1]; delta input; loads input size=[2 1]; wf output; wr output; Fxf output; Fxr output; diag output size=[32 1]; valid output; repair_cfg parameter
function [alpha,wf,wr,Fxf,Fxr,diag,valid] = force_block(F,actual,delta,loads,repair_cfg)
% 轴力不做摩擦圆、被动方向或前轮可达角投影；CarSim轮胎力是实际响应。
% alpha采用未饱和小侧偏斜率反算，只生成前轮指令；原始Fx用于轮速/力矩前馈。
% 轮速逆解使用载荷尺度的连续正则化，避免Fy过零时突变；它不是轮胎力/力矩限幅。
V=actual(1);beta=actual(2);r=actual(3);vx=V*cos(beta);vy=V*sin(beta);
contact=atan2(vy+repair_cfg.a*r,vx);alpha=-F(2)/repair_cfg.Caf;
vxf=vx*cos(delta)+(vy+repair_cfg.a*r)*sin(delta);
vyf=-vx*sin(delta)+(vy+repair_cfg.a*r)*cos(delta);vyr=vy-repair_cfg.b*r;
ef=repair_cfg.force_eps_frac*repair_cfg.mu*loads(1);
er=repair_cfg.force_eps_frac*repair_cfg.mu*loads(2);
wf=(vxf-vyf*F(1)*F(2)/(F(2)^2+ef^2))/repair_cfg.Rw;
wr=(vx-vyr*F(3)*F(4)/(F(4)^2+er^2))/repair_cfg.Rw;
Fxf=F(1);Fxr=F(3);valid=all(isfinite([F;actual;delta;loads;alpha;wf;wr]));
body=zeros(3,1);diag=[F;F;zeros(4,1);body;contact-alpha;contact-alpha;ef;er; ...
    ef^2/(F(2)^2+ef^2);er^2/(F(4)^2+er^2);0;0;vxf;vyf;vx;vyr;F(4)*vyr; ...
    repair_cfg.mu*loads(1);repair_cfg.mu*loads(2);NaN;double(~valid)];
end
